simulink library "Suspension_Utilities"  (R2025a)
settings: Solver=VariableStepAuto  StartTime=0.0  StopTime=10.0  RelTol=1e-3
undefined symbols (not defined in the file or in its folder): Ac, Af, Ar, hp1, hp2, hp3, hp_in, hp_in_f_ua, hp_in_r_ua, hp_mount_subframe, hp_shk_frame, hp_spr_bot, hp_spr_top, hpb, hpf, hpo, hpx, hpz, Newton, Raphson, rotYAxis, SubframeConnection, Upper_Arm_to_Subframe, Visual, X, Y, Z
libraries: sm_lib x75, $bdroot x23, linkage_bushing_6DOF_lib x13, fl_lib x4, sharedtransformsys x3, linkage_bushing_5DOF_lib x2, nesl_utility x1
(part 3 of 3)

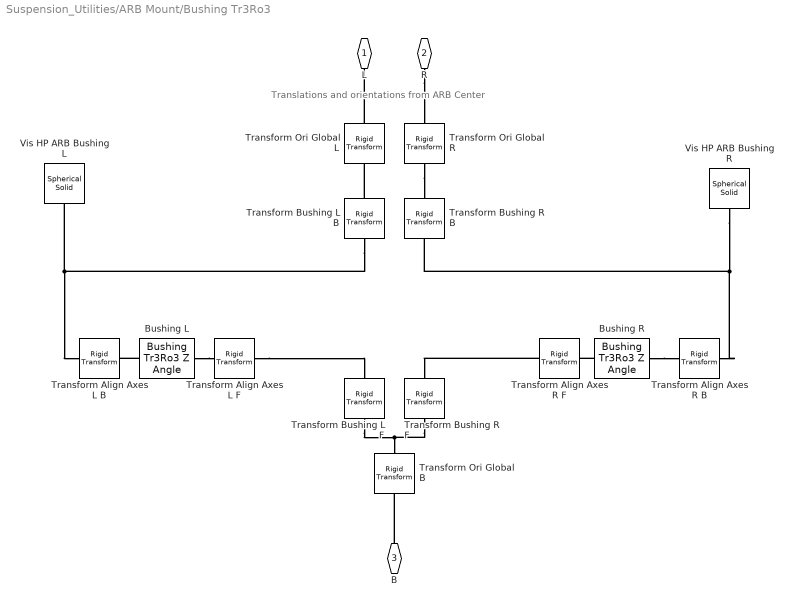
== system Suspension_Utilities/ARB Mount/Bushing Tr3Ro3 ==
  note: Translations and orientations from ARB Center
  Bushing L : linkage_bushing_6DOF_lib/Bushing Tr3Ro3 Z Angle  VariantControl=Bushing_Tr3Ro3  checkbox_setTargets=off  leftOrRight=1  qOriZ=Connection.qOriZ.Value  sprx=Connection.SpringX  spry=Connection.SpringY  sprz=Connection.SpringZ  damx=Connection.DamperX  damy=Connection.DamperY  damz=Connection.DamperZ  sprqx=Connection.SpringqX  sprqy=Connection.SpringqY  sprqz=Connection.SpringqZ  damqx=Connection.DamperqX  damqy=Connection.DamperqY  damqz=Connection.DamperqZ  shell_or=Visual.hp.rad*2  shell_len=Visual.hp.rad*2  shell_clr=Visual.BushingShell.clr  shell_opc=Visual.part.opc  sleeve_clr=Visual.Bushing.clr  sleeve_opc=Visual.part.opc
  Bushing R : linkage_bushing_6DOF_lib/Bushing Tr3Ro3 Z Angle  VariantControl=Bushing_Tr3Ro3  checkbox_setTargets=off  leftOrRight=-1  qOriZ=Connection.qOriZ.Value  sprx=Connection.SpringX  spry=Connection.SpringY  sprz=Connection.SpringZ  damx=Connection.DamperX  damy=Connection.DamperY  damz=Connection.DamperZ  sprqx=Connection.SpringqX  sprqy=Connection.SpringqY  sprqz=Connection.SpringqZ  damqx=Connection.DamperqX  damqy=Connection.DamperqY  damqz=Connection.DamperqZ  shell_or=Visual.hp.rad*2  shell_len=Visual.hp.rad*2  shell_clr=Visual.BushingShell.clr  shell_opc=Visual.part.opc  sleeve_clr=Visual.Bushing.clr  sleeve_opc=Visual.part.opc
  Transform Align Axes L B : sm_lib/Frames and Transforms/Rigid Transform  RotationMethod=RotationSequence  FollAlignAxisA=+X  BaseAlignAxisA=+Y  FollAlignAxisB=+Y  BaseAlignAxisB=+Z  RotationStandardAxis=+Z  RotationAngle=90  RotationAngleUnits=deg  RotationArbitraryAxis=[0 0 1]  RotationSequenceAxes=FollowerAxes  RotationSequence=XZX  RotationSequenceAngles=[90 0 0]  RotationSequenceAnglesUnits=deg  RotationMatrix=[1 0 0; 0 1 0; 0 0 1]  Quaternion=[1 0 0 0]  TranslationMethod=None  TranslationCartesianOffset=[0 0 0]  TranslationCartesianOffsetUnits=m  TranslationStandardAxis=+Z  TranslationStandardOffset=0  TranslationStandardOffsetUnits=m  TranslationROffset=0  TranslationROffsetUnits=m  TranslationThetaOffset=0  TranslationThetaOffsetUnits=deg  TranslationZOffset=0  TranslationZOffsetUnits=m
  Transform Align Axes L F : sm_lib/Frames and Transforms/Rigid Transform  RotationMethod=RotationSequence  FollAlignAxisA=+X  BaseAlignAxisA=+Y  FollAlignAxisB=+Y  BaseAlignAxisB=+Z  RotationStandardAxis=+Z  RotationAngle=90  RotationAngleUnits=deg  RotationArbitraryAxis=[0 0 1]  RotationSequenceAxes=FollowerAxes  RotationSequence=XZX  RotationSequenceAngles=[90 0 0]  RotationSequenceAnglesUnits=deg  RotationMatrix=[1 0 0; 0 1 0; 0 0 1]  Quaternion=[1 0 0 0]  TranslationMethod=None  TranslationCartesianOffset=[0 0 0]  TranslationCartesianOffsetUnits=m  TranslationStandardAxis=+Z  TranslationStandardOffset=0  TranslationStandardOffsetUnits=m  TranslationROffset=0  TranslationROffsetUnits=m  TranslationThetaOffset=0  TranslationThetaOffsetUnits=deg  TranslationZOffset=0  TranslationZOffsetUnits=m
  Transform Align Axes R B : sm_lib/Frames and Transforms/Rigid Transform  RotationMethod=RotationSequence  FollAlignAxisA=+X  BaseAlignAxisA=+Y  FollAlignAxisB=+Y  BaseAlignAxisB=+Z  RotationStandardAxis=+Z  RotationAngle=90  RotationAngleUnits=deg  RotationArbitraryAxis=[0 0 1]  RotationSequenceAxes=FollowerAxes  RotationSequence=XZX  RotationSequenceAngles=[90 0 0]  RotationSequenceAnglesUnits=deg  RotationMatrix=[1 0 0; 0 1 0; 0 0 1]  Quaternion=[1 0 0 0]  TranslationMethod=None  TranslationCartesianOffset=[0 0 0]  TranslationCartesianOffsetUnits=m  TranslationStandardAxis=+Z  TranslationStandardOffset=0  TranslationStandardOffsetUnits=m  TranslationROffset=0  TranslationROffsetUnits=m  TranslationThetaOffset=0  TranslationThetaOffsetUnits=deg  TranslationZOffset=0  TranslationZOffsetUnits=m
  Transform Align Axes R F : sm_lib/Frames and Transforms/Rigid Transform  RotationMethod=RotationSequence  FollAlignAxisA=+X  BaseAlignAxisA=+Y  FollAlignAxisB=+Y  BaseAlignAxisB=+Z  RotationStandardAxis=+Z  RotationAngle=90  RotationAngleUnits=deg  RotationArbitraryAxis=[0 0 1]  RotationSequenceAxes=FollowerAxes  RotationSequence=XZX  RotationSequenceAngles=[90 0 0]  RotationSequenceAnglesUnits=deg  RotationMatrix=[1 0 0; 0 1 0; 0 0 1]  Quaternion=[1 0 0 0]  TranslationMethod=None  TranslationCartesianOffset=[0 0 0]  TranslationCartesianOffsetUnits=m  TranslationStandardAxis=+Z  TranslationStandardOffset=0  TranslationStandardOffsetUnits=m  TranslationROffset=0  TranslationROffsetUnits=m  TranslationThetaOffset=0  TranslationThetaOffsetUnits=deg  TranslationZOffset=0  TranslationZOffsetUnits=m
  Transform Bushing L B : sm_lib/Frames and Transforms/Rigid Transform  RotationMethod=None  FollAlignAxisA=+X  BaseAlignAxisA=+Y  FollAlignAxisB=+Y  BaseAlignAxisB=+Z  RotationStandardAxis=+Z  RotationAngle=0.0  RotationAngleUnits=deg  RotationArbitraryAxis=[0 0 1]  RotationSequenceAxes=FollowerAxes  RotationSequence=XYX  RotationSequenceAngles=[0 0 0]  RotationSequenceAnglesUnits=deg  RotationMatrix=[1 0 0; 0 1 0; 0 0 1]  Quaternion=[1 0 0 0]  TranslationMethod=Cartesian  TranslationCartesianOffset=hp_mount_subframe-hp_in.*[1 0 1]  TranslationCartesianOffsetUnits=m  TranslationStandardAxis=+Z  TranslationStandardOffset=0  TranslationStandardOffsetUnits=m  TranslationROffset=0  TranslationROffsetUnits=m  TranslationThetaOffset=0  TranslationThetaOffsetUnits=deg  TranslationZOffset=0  TranslationZOffsetUnits=m
  Transform Bushing L F : sm_lib/Frames and Transforms/Rigid Transform  RotationMethod=None  FollAlignAxisA=+X  BaseAlignAxisA=+Y  FollAlignAxisB=+Y  BaseAlignAxisB=+Z  RotationStandardAxis=+Z  RotationAngle=0.0  RotationAngleUnits=deg  RotationArbitraryAxis=[0 0 1]  RotationSequenceAxes=FollowerAxes  RotationSequence=XYX  RotationSequenceAngles=[0 0 0]  RotationSequenceAnglesUnits=deg  RotationMatrix=[1 0 0; 0 1 0; 0 0 1]  Quaternion=[1 0 0 0]  TranslationMethod=Cartesian  TranslationCartesianOffset=hp_mount_subframe-hp_in.*[1 0 1]  TranslationCartesianOffsetUnits=m  TranslationStandardAxis=+Z  TranslationStandardOffset=0  TranslationStandardOffsetUnits=m  TranslationROffset=0  TranslationROffsetUnits=m  TranslationThetaOffset=0  TranslationThetaOffsetUnits=deg  TranslationZOffset=0  TranslationZOffsetUnits=m
  Transform Bushing R B : sm_lib/Frames and Transforms/Rigid Transform  RotationMethod=None  FollAlignAxisA=+X  BaseAlignAxisA=+Y  FollAlignAxisB=+Y  BaseAlignAxisB=+Z  RotationStandardAxis=+Z  RotationAngle=0.0  RotationAngleUnits=deg  RotationArbitraryAxis=[0 0 1]  RotationSequenceAxes=FollowerAxes  RotationSequence=XYX  RotationSequenceAngles=[0 0 0]  RotationSequenceAnglesUnits=deg  RotationMatrix=[1 0 0; 0 1 0; 0 0 1]  Quaternion=[1 0 0 0]  TranslationMethod=Cartesian  TranslationCartesianOffset=hp_mount_subframe.*[1 -1 1]-hp_in.*[1 0 1]  TranslationCartesianOffsetUnits=m  TranslationStandardAxis=+Z  TranslationStandardOffset=0  TranslationStandardOffsetUnits=m  TranslationROffset=0  TranslationROffsetUnits=m  TranslationThetaOffset=0  TranslationThetaOffsetUnits=deg  TranslationZOffset=0  TranslationZOffsetUnits=m
  Transform Bushing R F : sm_lib/Frames and Transforms/Rigid Transform  RotationMethod=None  FollAlignAxisA=+X  BaseAlignAxisA=+Y  FollAlignAxisB=+Y  BaseAlignAxisB=+Z  RotationStandardAxis=+Z  RotationAngle=0.0  RotationAngleUnits=deg  RotationArbitraryAxis=[0 0 1]  RotationSequenceAxes=FollowerAxes  RotationSequence=XYX  RotationSequenceAngles=[0 0 0]  RotationSequenceAnglesUnits=deg  RotationMatrix=[1 0 0; 0 1 0; 0 0 1]  Quaternion=[1 0 0 0]  TranslationMethod=Cartesian  TranslationCartesianOffset=hp_mount_subframe.*[1 -1 1]-hp_in.*[1 0 1]  TranslationCartesianOffsetUnits=m  TranslationStandardAxis=+Z  TranslationStandardOffset=0  TranslationStandardOffsetUnits=m  TranslationROffset=0  TranslationROffsetUnits=m  TranslationThetaOffset=0  TranslationThetaOffsetUnits=deg  TranslationZOffset=0  TranslationZOffsetUnits=m
  Transform Ori Global B : sm_lib/Frames and Transforms/Rigid Transform  RotationMethod=StandardAxis  FollAlignAxisA=+X  BaseAlignAxisA=+Y  FollAlignAxisB=+Y  BaseAlignAxisB=+Z  RotationStandardAxis=+X  RotationAngle=90  RotationAngleUnits=deg  RotationArbitraryAxis=[0 0 1]  RotationSequenceAxes=FollowerAxes  RotationSequence=XYX  RotationSequenceAngles=[0 0 0]  RotationSequenceAnglesUnits=deg  RotationMatrix=[1 0 0; 0 1 0; 0 0 1]  Quaternion=[1 0 0 0]  TranslationMethod=None  TranslationCartesianOffset=[0 0 0]  TranslationCartesianOffsetUnits=m  TranslationStandardAxis=+Z  TranslationStandardOffset=0  TranslationStandardOffsetUnits=m  TranslationROffset=0  TranslationROffsetUnits=m  TranslationThetaOffset=0  TranslationThetaOffsetUnits=deg  TranslationZOffset=0  TranslationZOffsetUnits=m
  Transform Ori Global L : sm_lib/Frames and Transforms/Rigid Transform  RotationMethod=StandardAxis  FollAlignAxisA=+X  BaseAlignAxisA=+Y  FollAlignAxisB=+Y  BaseAlignAxisB=+Z  RotationStandardAxis=+X  RotationAngle=90  RotationAngleUnits=deg  RotationArbitraryAxis=[0 0 1]  RotationSequenceAxes=FollowerAxes  RotationSequence=XYX  RotationSequenceAngles=[0 0 0]  RotationSequenceAnglesUnits=deg  RotationMatrix=[1 0 0; 0 1 0; 0 0 1]  Quaternion=[1 0 0 0]  TranslationMethod=None  TranslationCartesianOffset=[0 0 0]  TranslationCartesianOffsetUnits=m  TranslationStandardAxis=+Z  TranslationStandardOffset=0  TranslationStandardOffsetUnits=m  TranslationROffset=0  TranslationROffsetUnits=m  TranslationThetaOffset=0  TranslationThetaOffsetUnits=deg  TranslationZOffset=0  TranslationZOffsetUnits=m
  Transform Ori Global R : sm_lib/Frames and Transforms/Rigid Transform  RotationMethod=StandardAxis  FollAlignAxisA=+X  BaseAlignAxisA=+Y  FollAlignAxisB=+Y  BaseAlignAxisB=+Z  RotationStandardAxis=+X  RotationAngle=90  RotationAngleUnits=deg  RotationArbitraryAxis=[0 0 1]  RotationSequenceAxes=FollowerAxes  RotationSequence=XYX  RotationSequenceAngles=[0 0 0]  RotationSequenceAnglesUnits=deg  RotationMatrix=[1 0 0; 0 1 0; 0 0 1]  Quaternion=[1 0 0 0]  TranslationMethod=None  TranslationCartesianOffset=[0 0 0]  TranslationCartesianOffsetUnits=m  TranslationStandardAxis=+Z  TranslationStandardOffset=0  TranslationStandardOffsetUnits=m  TranslationROffset=0  TranslationROffsetUnits=m  TranslationThetaOffset=0  TranslationThetaOffsetUnits=deg  TranslationZOffset=0  TranslationZOffsetUnits=m
  Vis HP ARB Bushing L : sm_lib/Body Elements/Spherical Solid  SphereRadius=rad_hp  SphereRadiusUnits=m  ExportEntireGeometry=off  InertiaType=CalculateFromGeometry  BasedOnType=Density  Density=1000  DensityUnits=kg/m^3  Mass=1  MassUnits=kg  CenterOfMass=[0 0 0]  CenterOfMassUnits=m  MomentsOfInertia=[1 1 1]  MomentsOfInertiaUnits=kg*m^2  ProductsOfInertia=[0 0 0]  ProductsOfInertiaUnits=kg*m^2  GraphicType=FromGeometry  MarkerShape=Sphere  MarkerSize=10  GraphicVisPropType=SimpleVisualProperties  GraphicDiffuseColor=clr_hp  GraphicOpacity=opc_hp  GraphicSpecularColor=[0.5 0.5 0.5 1.0]  GraphicAmbientColor=[0.15 0.15 0.15 1.0]  GraphicEmissiveColor=[0.0 0.0 0.0 1.0]  GraphicShininess=75  DoExposeReferenceFrame=on  SerializedFrames=<Frames/>
  Vis HP ARB Bushing R : sm_lib/Body Elements/Spherical Solid  SphereRadius=rad_hp  SphereRadiusUnits=m  ExportEntireGeometry=off  InertiaType=CalculateFromGeometry  BasedOnType=Density  Density=1000  DensityUnits=kg/m^3  Mass=1  MassUnits=kg  CenterOfMass=[0 0 0]  CenterOfMassUnits=m  MomentsOfInertia=[1 1 1]  MomentsOfInertiaUnits=kg*m^2  ProductsOfInertia=[0 0 0]  ProductsOfInertiaUnits=kg*m^2  GraphicType=FromGeometry  MarkerShape=Sphere  MarkerSize=10  GraphicVisPropType=SimpleVisualProperties  GraphicDiffuseColor=clr_hp  GraphicOpacity=opc_hp  GraphicSpecularColor=[0.5 0.5 0.5 1.0]  GraphicAmbientColor=[0.15 0.15 0.15 1.0]  GraphicEmissiveColor=[0.0 0.0 0.0 1.0]  GraphicShininess=75  DoExposeReferenceFrame=on  SerializedFrames=<Frames/>
  L : PMIOPort  Side=Right
  R : PMIOPort  Port=2  Side=Right
  B : PMIOPort  Port=3  Side=Left
  connections:
  Transform Bushing L B/LConn1 -- Transform Ori Global L/RConn1
  Transform Ori Global L/LConn1 -- L/RConn1
  Transform Align Axes L F/LConn1 -- Transform Bushing L F/RConn1
  Transform Ori Global B/RConn1 -- Transform Bushing R F/LConn1 -- Transform Bushing L F/LConn1
  Transform Align Axes R F/LConn1 -- Transform Bushing R F/RConn1
  B/RConn1 -- Transform Ori Global B/LConn1
  Transform Ori Global R/RConn1 -- Transform Bushing R B/LConn1
  Vis HP ARB Bushing L/RConn1 -- Transform Align Axes L B/LConn1 -- Transform Bushing L B/RConn1
  Transform Bushing R B/RConn1 -- Transform Align Axes R B/LConn1 -- Vis HP ARB Bushing R/RConn1
  R/RConn1 -- Transform Ori Global R/LConn1
  Bushing R/LConn1 -- Transform Align Axes R B/RConn1
  Bushing R/RConn1 -- Transform Align Axes R F/RConn1
  Bushing L/LConn1 -- Transform Align Axes L B/RConn1
  Bushing L/RConn1 -- Transform Align Axes L F/RConn1

== system Suspension_Utilities/ARB Mount/Rigid 1Rev ==
  Revolute ARB Mount : sm_lib/Joints/Revolute Joint  JointMode=Normal  CompositeWrenchDir=FollowerOnBase  CompositeWrenchFrame=BaseFrame  SenseConstraintForce=off  SenseConstraintTorque=off  SenseTotalForce=off  SenseTotalTorque=off  PositionTargetSpecify=on  PositionTargetPriority=Low  PositionTargetValue=0  PositionTargetValueUnits=deg  VelocityTargetSpecify=off  VelocityTargetPriority=High  VelocityTargetValue=0  VelocityTargetValueUnits=deg/s  EquilibriumPosition=0  EquilibriumPositionUnits=deg  SpringStiffness=0  SpringStiffnessUnits=N*m/deg  DampingCoefficient=0  DampingCoefficientUnits=N*m/(deg/s)  LowerLimitSpecify=off  LowerLimitBound=-90  LowerLimitBoundUnits=deg  LowerLimitStiffness=1e4  LowerLimitStiffnessUnits=N*m/deg  LowerLimitDamping=10  LowerLimitDampingUnits=N*m/(deg/s)  LowerLimitTransitionRegionWidth=0.1  LowerLimitTransitionRegionWidthUnits=deg  UpperLimitSpecify=off  UpperLimitBound=90  UpperLimitBoundUnits=deg  UpperLimitStiffness=1e4  UpperLimitStiffnessUnits=N*m/deg  UpperLimitDamping=10  UpperLimitDampingUnits=N*m/(deg/s)  UpperLimitTransitionRegionWidth=0.1  UpperLimitTransitionRegionWidthUnits=deg  TorqueActuationMode=NoTorque  MotionActuationMode=ComputedMotion  SensePosition=off  SenseVelocity=off  SenseAcceleration=off  SenseTorqueForce=off  SenseLowerLimitTorqueForce=off  SenseUpperLimitTorqueForce=off
  L : PMIOPort  Side=Right
  R : PMIOPort  Port=2  Side=Right
  B : PMIOPort  Port=3  Side=Left
  connections:
  Revolute ARB Mount/LConn1 -- B/RConn1
  Revolute ARB Mount/RConn1 -- R/RConn1

== system Suspension_Utilities/Arm to Subframe Revolute/Bushing Ax3 ==
  Bushing Af : linkage_bushing_6DOF_lib/Bushing Ax3  VariantControl=Bushing_Ax3  checkbox_setTargets=on  leftOrRight=rhs_y  hp_j=hp_f  hp_z=Connection.sFAxialOrientationZ.Value  hp_x=Connection.sFAxialOrientationX.Value  AxisAttachment=Connection.AxisAttachment.class.Value  sprx=Connection.FSpringX  spry=Connection.FSpringY  sprz=Connection.FSpringZ  damx=Connection.FDamperX  damy=Connection.FDamperY  damz=Connection.FDamperZ  shell_or=Visual.hp.rad*2  shell_len=Visual.hp.rad*2  shell_clr=Visual.BushingShell.clr  shell_opc=Visual.part.opc  sleeve_clr=Visual.Bushing.clr  sleeve_opc=Visual.part.opc
  Bushing Ar : linkage_bushing_6DOF_lib/Bushing Ax3  VariantControl=Bushing_Ax3  checkbox_setTargets=off  leftOrRight=rhs_y  hp_j=hp_r  hp_z=Connection.sRAxialOrientationZ.Value  hp_x=Connection.sRAxialOrientationX.Value  AxisAttachment=Connection.AxisAttachment.class.Value  sprx=Connection.RSpringX  spry=Connection.RSpringY  sprz=Connection.RSpringZ  damx=Connection.RDamperX  damy=Connection.RDamperY  damz=Connection.RDamperZ  shell_or=Visual.hp.rad*2  shell_len=Visual.hp.rad*2  shell_clr=Visual.BushingShell.clr  shell_opc=Visual.part.opc  sleeve_clr=Visual.Bushing.clr  sleeve_opc=Visual.part.opc
  Simscape Bus : SimscapeBus  HierarchyStrings=Af;Ac;Ar
  Simscape Bus1 : SimscapeBus  HierarchyStrings=Af;Ac;Ar
  Terminator UAc Body : $bdroot/Terminator  SystemSampleTime=-1  VariantActivationTime=update diagram  EmptyChoice=off  PassThrough=off  PassThroughVariantControl=(default)  EmptyChoiceVariantControl=(default)  AllowFlexibleInterface=on  Latency=0  AutoFrameSizeCalculation=off
  Terminator UAc Chassis : $bdroot/Terminator  SystemSampleTime=-1  VariantActivationTime=update diagram  EmptyChoice=off  PassThrough=off  PassThroughVariantControl=(default)  EmptyChoiceVariantControl=(default)  AllowFlexibleInterface=on  Latency=0  AutoFrameSizeCalculation=off
  F : PMIOPort  Side=Right
  " B" : PMIOPort  Port=2  Side=Left
  connections:
  Simscape Bus1/RConn1 -- F/RConn1
  Simscape Bus/RConn1 -- " B"/RConn1
  Bushing Af/LConn1 -- Simscape Bus/LConn1
  Bushing Ar/LConn1 -- Simscape Bus/LConn3
  Simscape Bus1/LConn1 -- Bushing Af/RConn1
  Simscape Bus1/LConn3 -- Bushing Ar/RConn1
  Terminator UAc Body/RConn1 -- Simscape Bus/LConn2
  Terminator UAc Chassis/RConn1 -- Simscape Bus1/LConn2

== system Suspension_Utilities/Arm to Subframe Revolute/Bushing AxRad ==
  Bushing Af : linkage_bushing_6DOF_lib/Bushing AxRad  VariantControl=Bushing_AxRad  checkbox_setTargets=on  leftOrRight=rhs_y  hp_j=hp_f  hp_z=hp_r  sprRad=Connection.RadialSpring  damRad=Connection.RadialDamper  sprAxi=Connection.AxialSpring  damAxi=Connection.AxialDamper  shell_or=Visual.hp.rad*2  shell_len=Visual.hp.rad*2  shell_clr=Visual.BushingShell.clr  shell_opc=Visual.part.opc  sleeve_clr=Visual.Bushing.clr  sleeve_opc=Visual.part.opc
  Bushing Ar : linkage_bushing_6DOF_lib/Bushing AxRad  VariantControl=Bushing_AxRad  checkbox_setTargets=off  leftOrRight=rhs_y  hp_j=hp_r  hp_z=hp_f  sprRad=Connection.RadialSpring  damRad=Connection.RadialDamper  sprAxi=Connection.AxialSpring  damAxi=Connection.AxialDamper  shell_or=Visual.hp.rad*2  shell_len=Visual.hp.rad*2  shell_clr=Visual.BushingShell.clr  shell_opc=Visual.part.opc  sleeve_clr=Visual.Bushing.clr  sleeve_opc=Visual.part.opc
  Simscape Bus : SimscapeBus  HierarchyStrings=Af;Ac;Ar
  Simscape Bus1 : SimscapeBus  HierarchyStrings=Af;Ac;Ar
  Terminator UAc Body : $bdroot/Terminator  SystemSampleTime=-1  VariantActivationTime=update diagram  EmptyChoice=off  PassThrough=off  PassThroughVariantControl=(default)  EmptyChoiceVariantControl=(default)  AllowFlexibleInterface=on  Latency=0  AutoFrameSizeCalculation=off
  Terminator UAc Chassis : $bdroot/Terminator  SystemSampleTime=-1  VariantActivationTime=update diagram  EmptyChoice=off  PassThrough=off  PassThroughVariantControl=(default)  EmptyChoiceVariantControl=(default)  AllowFlexibleInterface=on  Latency=0  AutoFrameSizeCalculation=off
  F : PMIOPort  Side=Right
  " B" : PMIOPort  Port=2  Side=Left
  connections:
  Terminator UAc Chassis/RConn1 -- Simscape Bus1/LConn2
  Terminator UAc Body/RConn1 -- Simscape Bus/LConn2
  Simscape Bus/RConn1 -- " B"/RConn1
  Simscape Bus1/RConn1 -- F/RConn1
  Bushing Af/LConn1 -- Simscape Bus/LConn1
  Bushing Af/RConn1 -- Simscape Bus1/LConn1
  Bushing Ar/LConn1 -- Simscape Bus/LConn3
  Bushing Ar/RConn1 -- Simscape Bus1/LConn3

== system Suspension_Utilities/Arm to Subframe Revolute/Bushing Tr3Ro3 ==
  Bushing Af : linkage_bushing_6DOF_lib/Bushing Tr3Ro3 2Pts  VariantControl=Bushing_Tr3Ro3  checkbox_setTargets=on  leftOrRight=rhs_y  hp_j=hp_f  hp_z=Connection.sFAxialOrientationZ.Value  hp_x=Connection.sFAxialOrientationX.Value  sprx=Connection.FSpringX  spry=Connection.FSpringY  sprz=Connection.FSpringZ  damx=Connection.FDamperX  damy=Connection.FDamperY  damz=Connection.FDamperZ  sprqx=Connection.FSpringqX  sprqy=Connection.FSpringqY  sprqz=Connection.FSpringqZ  damqx=Connection.FDamperqX  damqy=Connection.FDamperqY  damqz=Connection.FDamperqZ  shell_or=Visual.hp.rad*2  shell_len=Visual.hp.rad*2  shell_clr=Visual.BushingShell.clr  shell_opc=Visual.part.opc  sleeve_clr=Visual.Bushing.clr  sleeve_opc=Visual.part.opc
  Bushing Ar : linkage_bushing_6DOF_lib/Bushing Tr3Ro3 2Pts  VariantControl=Bushing_Tr3Ro3  checkbox_setTargets=off  leftOrRight=rhs_y  hp_j=hp_r  hp_z=Connection.sRAxialOrientationZ.Value  hp_x=Connection.sRAxialOrientationX.Value  sprx=Connection.RSpringX  spry=Connection.RSpringY  sprz=Connection.RSpringZ  damx=Connection.RDamperX  damy=Connection.RDamperY  damz=Connection.RDamperZ  sprqx=Connection.RSpringqX  sprqy=Connection.RSpringqY  sprqz=Connection.RSpringqZ  damqx=Connection.RDamperqX  damqy=Connection.RDamperqY  damqz=Connection.RDamperqZ  shell_or=Visual.hp.rad*2  shell_len=Visual.hp.rad*2  shell_clr=Visual.BushingShell.clr  shell_opc=Visual.part.opc  sleeve_clr=Visual.Bushing.clr  sleeve_opc=Visual.part.opc
  Simscape Bus : SimscapeBus  HierarchyStrings=Af;Ac;Ar
  Simscape Bus1 : SimscapeBus  HierarchyStrings=Af;Ac;Ar
  Terminator UAc Body : $bdroot/Terminator  SystemSampleTime=-1  VariantActivationTime=update diagram  EmptyChoice=off  PassThrough=off  PassThroughVariantControl=(default)  EmptyChoiceVariantControl=(default)  AllowFlexibleInterface=on  Latency=0  AutoFrameSizeCalculation=off
  Terminator UAc Chassis : $bdroot/Terminator  SystemSampleTime=-1  VariantActivationTime=update diagram  EmptyChoice=off  PassThrough=off  PassThroughVariantControl=(default)  EmptyChoiceVariantControl=(default)  AllowFlexibleInterface=on  Latency=0  AutoFrameSizeCalculation=off
  F : PMIOPort  Side=Right
  " B" : PMIOPort  Port=2  Side=Left
  connections:
  Terminator UAc Chassis/RConn1 -- Simscape Bus1/LConn2
  Terminator UAc Body/RConn1 -- Simscape Bus/LConn2
  Simscape Bus/RConn1 -- " B"/RConn1
  Simscape Bus1/RConn1 -- F/RConn1
  Bushing Af/LConn1 -- Simscape Bus/LConn1
  Bushing Af/RConn1 -- Simscape Bus1/LConn1
  Bushing Ar/RConn1 -- Simscape Bus1/LConn3
  Bushing Ar/LConn1 -- Simscape Bus/LConn3

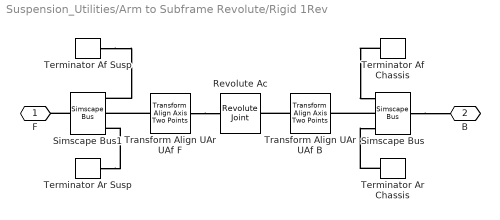
== system Suspension_Utilities/Arm to Subframe Revolute/Rigid 1Rev ==
  Revolute Ac : sm_lib/Joints/Revolute Joint  JointMode=Normal  CompositeWrenchDir=FollowerOnBase  CompositeWrenchFrame=BaseFrame  SenseConstraintForce=off  SenseConstraintTorque=off  SenseTotalForce=off  SenseTotalTorque=off  PositionTargetSpecify=on  PositionTargetPriority=Low  PositionTargetValue=0  PositionTargetValueUnits=deg  VelocityTargetSpecify=off  VelocityTargetPriority=High  VelocityTargetValue=0  VelocityTargetValueUnits=deg/s  EquilibriumPosition=0  EquilibriumPositionUnits=deg  SpringStiffness=0  SpringStiffnessUnits=N*m/deg  DampingCoefficient=0  DampingCoefficientUnits=N*m/(deg/s)  LowerLimitSpecify=off  LowerLimitBound=-90  LowerLimitBoundUnits=deg  LowerLimitStiffness=1e4  LowerLimitStiffnessUnits=N*m/deg  LowerLimitDamping=10  LowerLimitDampingUnits=N*m/(deg/s)  LowerLimitTransitionRegionWidth=0.1  LowerLimitTransitionRegionWidthUnits=deg  UpperLimitSpecify=off  UpperLimitBound=90  UpperLimitBoundUnits=deg  UpperLimitStiffness=1e4  UpperLimitStiffnessUnits=N*m/deg  UpperLimitDamping=10  UpperLimitDampingUnits=N*m/(deg/s)  UpperLimitTransitionRegionWidth=0.1  UpperLimitTransitionRegionWidthUnits=deg  TorqueActuationMode=NoTorque  MotionActuationMode=ComputedMotion  SensePosition=off  SenseVelocity=off  SenseAcceleration=off  SenseTorqueForce=off  SenseLowerLimitTorqueForce=off  SenseUpperLimitTorqueForce=off
  Simscape Bus : SimscapeBus  HierarchyStrings=Af;Ac;Ar
  Simscape Bus1 : SimscapeBus  HierarchyStrings=Af;Ac;Ar
  Terminator Af Chassis : $bdroot/Terminator  SystemSampleTime=-1  VariantActivationTime=update diagram  EmptyChoice=off  PassThrough=off  PassThroughVariantControl=(default)  EmptyChoiceVariantControl=(default)  AllowFlexibleInterface=on  Latency=0  AutoFrameSizeCalculation=off
  Terminator Af Susp : $bdroot/Terminator  SystemSampleTime=-1  VariantActivationTime=update diagram  EmptyChoice=off  PassThrough=off  PassThroughVariantControl=(default)  EmptyChoiceVariantControl=(default)  AllowFlexibleInterface=on  Latency=0  AutoFrameSizeCalculation=off
  Terminator Ar Chassis : $bdroot/Terminator  SystemSampleTime=-1  VariantActivationTime=update diagram  EmptyChoice=off  PassThrough=off  PassThroughVariantControl=(default)  EmptyChoiceVariantControl=(default)  AllowFlexibleInterface=on  Latency=0  AutoFrameSizeCalculation=off
  Terminator Ar Susp : $bdroot/Terminator  SystemSampleTime=-1  VariantActivationTime=update diagram  EmptyChoice=off  PassThrough=off  PassThroughVariantControl=(default)  EmptyChoiceVariantControl=(default)  AllowFlexibleInterface=on  Latency=0  AutoFrameSizeCalculation=off
  Transform Align UAr UAf B : $bdroot/Transform Align Axis Two Points  hp_b=hp_r.*rhs_hp  hp_t=hp_f.*rhs_hp  popup_f_axis=+Z
  Transform Align UAr UAf F : $bdroot/Transform Align Axis Two Points  hp_b=hp_r.*rhs_hp  hp_t=hp_f.*rhs_hp  popup_f_axis=+Z
  F : PMIOPort  Side=Right
  " B" : PMIOPort  Port=2  Side=Left
  connections:
  Transform Align UAr UAf F/LConn1 -- Simscape Bus1/LConn2
  Transform Align UAr UAf B/RConn1 -- Revolute Ac/LConn1
  Simscape Bus/LConn2 -- Transform Align UAr UAf B/LConn1
  Transform Align UAr UAf F/RConn1 -- Revolute Ac/RConn1
  Simscape Bus/RConn1 -- " B"/RConn1
  Simscape Bus1/RConn1 -- F/RConn1
  Terminator Af Susp/RConn1 -- Simscape Bus1/LConn1
  Terminator Ar Susp/RConn1 -- Simscape Bus1/LConn3
  Terminator Af Chassis/RConn1 -- Simscape Bus/LConn1
  Terminator Ar Chassis/RConn1 -- Simscape Bus/LConn3

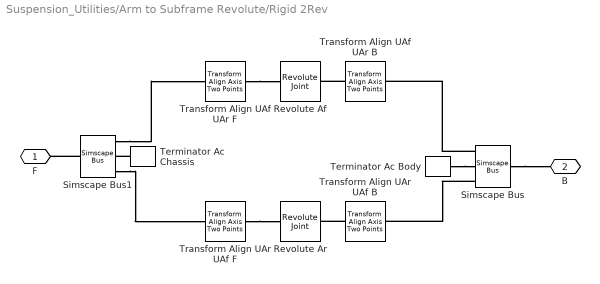
== system Suspension_Utilities/Arm to Subframe Revolute/Rigid 2Rev ==
  Revolute Af : sm_lib/Joints/Revolute Joint  JointMode=Normal  CompositeWrenchDir=FollowerOnBase  CompositeWrenchFrame=BaseFrame  SenseConstraintForce=off  SenseConstraintTorque=off  SenseTotalForce=off  SenseTotalTorque=off  PositionTargetSpecify=on  PositionTargetPriority=Low  PositionTargetValue=0  PositionTargetValueUnits=deg  VelocityTargetSpecify=off  VelocityTargetPriority=High  VelocityTargetValue=0  VelocityTargetValueUnits=deg/s  EquilibriumPosition=0  EquilibriumPositionUnits=deg  SpringStiffness=0  SpringStiffnessUnits=N*m/deg  DampingCoefficient=0  DampingCoefficientUnits=N*m/(deg/s)  LowerLimitSpecify=off  LowerLimitBound=-90  LowerLimitBoundUnits=deg  LowerLimitStiffness=1e4  LowerLimitStiffnessUnits=N*m/deg  LowerLimitDamping=10  LowerLimitDampingUnits=N*m/(deg/s)  LowerLimitTransitionRegionWidth=0.1  LowerLimitTransitionRegionWidthUnits=deg  UpperLimitSpecify=off  UpperLimitBound=90  UpperLimitBoundUnits=deg  UpperLimitStiffness=1e4  UpperLimitStiffnessUnits=N*m/deg  UpperLimitDamping=10  UpperLimitDampingUnits=N*m/(deg/s)  UpperLimitTransitionRegionWidth=0.1  UpperLimitTransitionRegionWidthUnits=deg  TorqueActuationMode=NoTorque  MotionActuationMode=ComputedMotion  SensePosition=off  SenseVelocity=off  SenseAcceleration=off  SenseTorqueForce=off  SenseLowerLimitTorqueForce=off  SenseUpperLimitTorqueForce=off
  Revolute Ar : sm_lib/Joints/Revolute Joint  JointMode=Normal  CompositeWrenchDir=FollowerOnBase  CompositeWrenchFrame=BaseFrame  SenseConstraintForce=off  SenseConstraintTorque=off  SenseTotalForce=off  SenseTotalTorque=off  PositionTargetSpecify=off  PositionTargetPriority=Low  PositionTargetValue=0  PositionTargetValueUnits=deg  VelocityTargetSpecify=off  VelocityTargetPriority=High  VelocityTargetValue=0  VelocityTargetValueUnits=deg/s  EquilibriumPosition=0  EquilibriumPositionUnits=deg  SpringStiffness=0  SpringStiffnessUnits=N*m/deg  DampingCoefficient=0  DampingCoefficientUnits=N*m/(deg/s)  LowerLimitSpecify=off  LowerLimitBound=-90  LowerLimitBoundUnits=deg  LowerLimitStiffness=1e4  LowerLimitStiffnessUnits=N*m/deg  LowerLimitDamping=10  LowerLimitDampingUnits=N*m/(deg/s)  LowerLimitTransitionRegionWidth=0.1  LowerLimitTransitionRegionWidthUnits=deg  UpperLimitSpecify=off  UpperLimitBound=90  UpperLimitBoundUnits=deg  UpperLimitStiffness=1e4  UpperLimitStiffnessUnits=N*m/deg  UpperLimitDamping=10  UpperLimitDampingUnits=N*m/(deg/s)  UpperLimitTransitionRegionWidth=0.1  UpperLimitTransitionRegionWidthUnits=deg  TorqueActuationMode=NoTorque  MotionActuationMode=ComputedMotion  SensePosition=off  SenseVelocity=off  SenseAcceleration=off  SenseTorqueForce=off  SenseLowerLimitTorqueForce=off  SenseUpperLimitTorqueForce=off
  Simscape Bus : SimscapeBus  HierarchyStrings=Af;Ac;Ar
  Simscape Bus1 : SimscapeBus  HierarchyStrings=Af;Ac;Ar
  Terminator Ac Body : $bdroot/Terminator  SystemSampleTime=-1  VariantActivationTime=update diagram  EmptyChoice=off  PassThrough=off  PassThroughVariantControl=(default)  EmptyChoiceVariantControl=(default)  AllowFlexibleInterface=on  Latency=0  AutoFrameSizeCalculation=off
  Terminator Ac Chassis : $bdroot/Terminator  SystemSampleTime=-1  VariantActivationTime=update diagram  EmptyChoice=off  PassThrough=off  PassThroughVariantControl=(default)  EmptyChoiceVariantControl=(default)  AllowFlexibleInterface=on  Latency=0  AutoFrameSizeCalculation=off
  Transform Align UAf UAr B : $bdroot/Transform Align Axis Two Points  hp_b=hp_f.*rhs_hp  hp_t=hp_r.*rhs_hp  popup_f_axis=-Z
  Transform Align UAf UAr F : $bdroot/Transform Align Axis Two Points  hp_b=hp_f.*rhs_hp  hp_t=hp_r.*rhs_hp  popup_f_axis=-Z
  Transform Align UAr UAf B : $bdroot/Transform Align Axis Two Points  hp_b=hp_r.*rhs_hp  hp_t=hp_f.*rhs_hp  popup_f_axis=+Z
  Transform Align UAr UAf F : $bdroot/Transform Align Axis Two Points  hp_b=hp_r.*rhs_hp  hp_t=hp_f.*rhs_hp  popup_f_axis=+Z
  F : PMIOPort  Side=Right
  " B" : PMIOPort  Port=2  Side=Left
  connections:
  Simscape Bus1/LConn1 -- Transform Align UAf UAr F/LConn1
  Transform Align UAr UAf F/RConn1 -- Revolute Ar/RConn1
  Transform Align UAr UAf B/RConn1 -- Revolute Ar/LConn1
  Transform Align UAf UAr F/RConn1 -- Revolute Af/RConn1
  Transform Align UAf UAr B/RConn1 -- Revolute Af/LConn1
  Terminator Ac Body/RConn1 -- Simscape Bus/LConn2
  Terminator Ac Chassis/RConn1 -- Simscape Bus1/LConn2
  Simscape Bus1/RConn1 -- F/RConn1
  Simscape Bus/RConn1 -- " B"/RConn1
  Simscape Bus/LConn1 -- Transform Align UAf UAr B/LConn1
  Simscape Bus/LConn3 -- Transform Align UAr UAf B/LConn1
  Simscape Bus1/LConn3 -- Transform Align UAr UAf F/LConn1

== system Suspension_Utilities/Arm to Subframe Universal/Rigid UJ ==
  Transform Align Y Up In : sm_lib/Frames and Transforms/Rigid Transform  RotationMethod=StandardAxis  FollAlignAxisA=+X  BaseAlignAxisA=+Y  FollAlignAxisB=+Y  BaseAlignAxisB=+Z  RotationStandardAxis=+X  RotationAngle=90  RotationAngleUnits=deg  RotationArbitraryAxis=[0 0 1]  RotationSequenceAxes=FollowerAxes  RotationSequence=XYX  RotationSequenceAngles=[0 0 0]  RotationSequenceAnglesUnits=deg  RotationMatrix=[1 0 0; 0 1 0; 0 0 1]  Quaternion=[1 0 0 0]  TranslationMethod=None  TranslationCartesianOffset=[0 0 0]  TranslationCartesianOffsetUnits=m  TranslationStandardAxis=+Z  TranslationStandardOffset=0  TranslationStandardOffsetUnits=m  TranslationROffset=0  TranslationROffsetUnits=m  TranslationThetaOffset=0  TranslationThetaOffsetUnits=deg  TranslationZOffset=0  TranslationZOffsetUnits=m
  Transform Align Y Up Out : sm_lib/Frames and Transforms/Rigid Transform  RotationMethod=StandardAxis  FollAlignAxisA=+X  BaseAlignAxisA=+Y  FollAlignAxisB=+Y  BaseAlignAxisB=+Z  RotationStandardAxis=+X  RotationAngle=90  RotationAngleUnits=deg  RotationArbitraryAxis=[0 0 1]  RotationSequenceAxes=FollowerAxes  RotationSequence=XYX  RotationSequenceAngles=[0 0 0]  RotationSequenceAnglesUnits=deg  RotationMatrix=[1 0 0; 0 1 0; 0 0 1]  Quaternion=[1 0 0 0]  TranslationMethod=None  TranslationCartesianOffset=[0 0 0]  TranslationCartesianOffsetUnits=m  TranslationStandardAxis=+Z  TranslationStandardOffset=0  TranslationStandardOffsetUnits=m  TranslationROffset=0  TranslationROffsetUnits=m  TranslationThetaOffset=0  TranslationThetaOffsetUnits=deg  TranslationZOffset=0  TranslationZOffsetUnits=m
  Universal Joint : sm_lib/Joints/Universal Joint  JointMode=Normal  CompositeWrenchDir=FollowerOnBase  CompositeWrenchFrame=BaseFrame  SenseConstraintForce=off  SenseConstraintTorque=off  SenseTotalForce=off  SenseTotalTorque=off  RxPositionTargetSpecify=on  RxPositionTargetPriority=Low  RxPositionTargetValue=0  RxPositionTargetValueUnits=deg  RxVelocityTargetSpecify=off  RxVelocityTargetPriority=High  RxVelocityTargetValue=0  RxVelocityTargetValueUnits=deg/s  RxEquilibriumPosition=0  RxEquilibriumPositionUnits=deg  RxSpringStiffness=0  RxSpringStiffnessUnits=N*m/deg  RxDampingCoefficient=0  RxDampingCoefficientUnits=N*m/(deg/s)  RxLowerLimitSpecify=off  RxLowerLimitBound=-90  RxLowerLimitBoundUnits=deg  RxLowerLimitStiffness=1e4  RxLowerLimitStiffnessUnits=N*m/deg  RxLowerLimitDamping=10  RxLowerLimitDampingUnits=N*m/(deg/s)  RxLowerLimitTransitionRegionWidth=0.1  RxLowerLimitTransitionRegionWidthUnits=deg  RxUpperLimitSpecify=off  RxUpperLimitBound=90  RxUpperLimitBoundUnits=deg  RxUpperLimitStiffness=1e4  RxUpperLimitStiffnessUnits=N*m/deg  RxUpperLimitDamping=10  RxUpperLimitDampingUnits=N*m/(deg/s)  RxUpperLimitTransitionRegionWidth=0.1  RxUpperLimitTransitionRegionWidthUnits=deg  RxTorqueActuationMode=NoTorque  RxMotionActuationMode=ComputedMotion  RxSensePosition=off  RxSenseVelocity=off  RxSenseAcceleration=off  RxSenseTorqueForce=off  RxSenseLowerLimitTorqueForce=off  RxSenseUpperLimitTorqueForce=off  RyPositionTargetSpecify=on  RyPositionTargetPriority=High  RyPositionTargetValue=0  RyPositionTargetValueUnits=deg  RyVelocityTargetSpecify=off  RyVelocityTargetPriority=High  RyVelocityTargetValue=0  RyVelocityTargetValueUnits=deg/s  RyEquilibriumPosition=0  RyEquilibriumPositionUnits=deg  RySpringStiffness=0  RySpringStiffnessUnits=N*m/deg  RyDampingCoefficient=0  RyDampingCoefficientUnits=N*m/(deg/s)  RyLowerLimitSpecify=off  RyLowerLimitBound=-90  RyLowerLimitBoundUnits=deg  RyLowerLimitStiffness=1e4  RyLowerLimitStiffnessUnits=N*m/deg  RyLowerLimitDamping=10  RyLowerLimitDampingUnits=N*m/(deg/s)  RyLowerLimitTransitionRegionWidth=0.1  RyLowerLimitTransitionRegionWidthUnits=deg  RyUpperLimitSpecify=off  RyUpperLimitBound=90  RyUpperLimitBoundUnits=deg  RyUpperLimitStiffness=1e4  RyUpperLimitStiffnessUnits=N*m/deg  RyUpperLimitDamping=10  RyUpperLimitDampingUnits=N*m/(deg/s)  RyUpperLimitTransitionRegionWidth=0.1  RyUpperLimitTransitionRegionWidthUnits=deg  RyTorqueActuationMode=NoTorque  RyMotionActuationMode=ComputedMotion  RySensePosition=off  RySenseVelocity=off  RySenseAcceleration=off  RySenseTorqueForce=off  RySenseLowerLimitTorqueForce=off  RySenseUpperLimitTorqueForce=off
  F : PMIOPort  Side=Right
  B : PMIOPort  Port=2  Side=Left
  connections:
  B/RConn1 -- Transform Align Y Up In/LConn1
  F/RConn1 -- Transform Align Y Up Out/LConn1
  Transform Align Y Up Out/RConn1 -- Universal Joint/RConn1
  Transform Align Y Up In/RConn1 -- Universal Joint/LConn1

== system Suspension_Utilities/Bushing Align 2Pts Gimbal/Rigid Gimbal ==
  Gimbal HP Spring : sm_lib/Joints/Gimbal Joint  JointMode=Normal  CompositeWrenchDir=FollowerOnBase  CompositeWrenchFrame=BaseFrame  SenseConstraintForce=off  SenseConstraintTorque=off  SenseTotalForce=off  SenseTotalTorque=off  RxPositionTargetSpecify=off  RxPositionTargetPriority=Low  RxPositionTargetValue=0  RxPositionTargetValueUnits=deg  RxVelocityTargetSpecify=off  RxVelocityTargetPriority=High  RxVelocityTargetValue=0  RxVelocityTargetValueUnits=deg/s  RxEquilibriumPosition=0  RxEquilibriumPositionUnits=deg  RxSpringStiffness=0  RxSpringStiffnessUnits=N*m/deg  RxDampingCoefficient=0  RxDampingCoefficientUnits=N*m/(deg/s)  RxLowerLimitSpecify=off  RxLowerLimitBound=-90  RxLowerLimitBoundUnits=deg  RxLowerLimitStiffness=1e4  RxLowerLimitStiffnessUnits=N*m/deg  RxLowerLimitDamping=10  RxLowerLimitDampingUnits=N*m/(deg/s)  RxLowerLimitTransitionRegionWidth=0.1  RxLowerLimitTransitionRegionWidthUnits=deg  RxUpperLimitSpecify=off  RxUpperLimitBound=90  RxUpperLimitBoundUnits=deg  RxUpperLimitStiffness=1e4  RxUpperLimitStiffnessUnits=N*m/deg  RxUpperLimitDamping=10  RxUpperLimitDampingUnits=N*m/(deg/s)  RxUpperLimitTransitionRegionWidth=0.1  RxUpperLimitTransitionRegionWidthUnits=deg  RxTorqueActuationMode=NoTorque  RxMotionActuationMode=ComputedMotion  RxSensePosition=off  RxSenseVelocity=off  RxSenseAcceleration=off  RxSenseTorqueForce=off  RxSenseLowerLimitTorqueForce=off  RxSenseUpperLimitTorqueForce=off  RyPositionTargetSpecify=off  RyPositionTargetPriority=High  RyPositionTargetValue=0  RyPositionTargetValueUnits=deg  RyVelocityTargetSpecify=off  RyVelocityTargetPriority=High  RyVelocityTargetValue=0  RyVelocityTargetValueUnits=deg/s  RyEquilibriumPosition=0  RyEquilibriumPositionUnits=deg  RySpringStiffness=0  RySpringStiffnessUnits=N*m/deg  RyDampingCoefficient=0  RyDampingCoefficientUnits=N*m/(deg/s)  RyLowerLimitSpecify=off  RyLowerLimitBound=-90  RyLowerLimitBoundUnits=deg  RyLowerLimitStiffness=1e4  RyLowerLimitStiffnessUnits=N*m/deg  RyLowerLimitDamping=10  RyLowerLimitDampingUnits=N*m/(deg/s)  RyLowerLimitTransitionRegionWidth=0.1  RyLowerLimitTransitionRegionWidthUnits=deg  RyUpperLimitSpecify=off  RyUpperLimitBound=90  RyUpperLimitBoundUnits=deg  RyUpperLimitStiffness=1e4  RyUpperLimitStiffnessUnits=N*m/deg  RyUpperLimitDamping=10  RyUpperLimitDampingUnits=N*m/(deg/s)  RyUpperLimitTransitionRegionWidth=0.1  RyUpperLimitTransitionRegionWidthUnits=deg  RyTorqueActuationMode=NoTorque  RyMotionActuationMode=ComputedMotion  RySensePosition=off  RySenseVelocity=off  RySenseAcceleration=off  RySenseTorqueForce=off  RySenseLowerLimitTorqueForce=off  RySenseUpperLimitTorqueForce=off  RzPositionTargetSpecify=off  RzPositionTargetPriority=High  RzPositionTargetValue=0  RzPositionTargetValueUnits=deg  RzVelocityTargetSpecify=off  RzVelocityTargetPriority=High  RzVelocityTargetValue=0  RzVelocityTargetValueUnits=deg/s  RzEquilibriumPosition=0  RzEquilibriumPositionUnits=deg  RzSpringStiffness=0  RzSpringStiffnessUnits=N*m/deg  RzDampingCoefficient=0  RzDampingCoefficientUnits=N*m/(deg/s)  RzLowerLimitSpecify=off  RzLowerLimitBound=-90  RzLowerLimitBoundUnits=deg  RzLowerLimitStiffness=1e4  RzLowerLimitStiffnessUnits=N*m/deg  RzLowerLimitDamping=10  RzLowerLimitDampingUnits=N*m/(deg/s)  RzLowerLimitTransitionRegionWidth=0.1  RzLowerLimitTransitionRegionWidthUnits=deg  RzUpperLimitSpecify=off  RzUpperLimitBound=90  RzUpperLimitBoundUnits=deg  RzUpperLimitStiffness=1e4  RzUpperLimitStiffnessUnits=N*m/deg  RzUpperLimitDamping=10  RzUpperLimitDampingUnits=N*m/(deg/s)  RzUpperLimitTransitionRegionWidth=0.1  RzUpperLimitTransitionRegionWidthUnits=deg  RzTorqueActuationMode=NoTorque  RzMotionActuationMode=ComputedMotion  RzSensePosition=off  RzSenseVelocity=off  RzSenseAcceleration=off  RzSenseTorqueForce=off  RzSenseLowerLimitTorqueForce=off  RzSenseUpperLimitTorqueForce=off
  F : PMIOPort  Side=Right
  B : PMIOPort  Port=2  Side=Left
  connections:
  Gimbal HP Spring/LConn1 -- B/RConn1
  Gimbal HP Spring/RConn1 -- F/RConn1

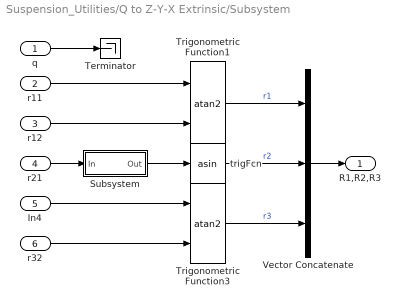
== system Suspension_Utilities/Q to Z-Y-X Extrinsic/Subsystem ==
  q : Inport
  r11 : Inport  Port=2
  r12 : Inport  Port=3
  r21 : Inport  Port=4
  In4 : Inport  Port=5
  r32 : Inport  Port=6
  Subsystem : Subsystem
  Terminator : Terminator
  Trigonometric Function1 : Trigonometry  Operator=atan2
  Trigonometric Function3 : Trigonometry  Operator=atan2
  Vector Concatenate : Concatenate  NumInputs=3
  trigFcn : Trigonometry  Operator=asin
  R1,R2,R3 : Outport  VectorParamsAs1DForOutWhenUnconnected=off
  wires:
  In4/1 -> Trigonometric Function3/1
  Trigonometric Function1/1 -> Vector Concatenate/1  "r1"
  Trigonometric Function3/1 -> Vector Concatenate/3  "r3"
  Subsystem/1(Out) -> trigFcn/1
  q/1 -> Terminator/1
  trigFcn/1 -> Vector Concatenate/2  "r2"
  r32/1 -> Trigonometric Function3/2
  r11/1 -> Trigonometric Function1/1
  r21/1 -> Subsystem/1(In)
  r12/1 -> Trigonometric Function1/2
  Vector Concatenate/1 -> R1,R2,R3/1

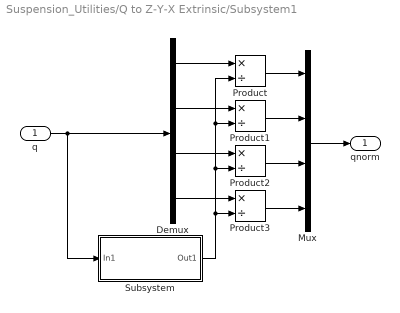
== system Suspension_Utilities/Q to Z-Y-X Extrinsic/Subsystem1 ==
  q : Inport  Unit=1
  Demux : Demux
  Mux : Mux
  Product{,1..3} (4 alike) : Product  Inputs=*/
  Subsystem : Subsystem
  qnorm : Outport  Unit=1  VectorParamsAs1DForOutWhenUnconnected=off
  wires:
  Product1/1 -> Mux/2
  Product3/1 -> Mux/4
  Demux/1 -> Product/1
  Subsystem/1(Out1) -> Product1/2, Product/2, Product2/2, Product3/2
  Mux/1 -> qnorm/1
  Product/1 -> Mux/1
  Demux/3 -> Product2/1
  Demux/4 -> Product3/1
  q/1 -> Demux/1, Subsystem/1(In1)
  Demux/2 -> Product1/1
  Product2/1 -> Mux/3

== system Suspension_Utilities/Shock to Subframe Gimbal/Rigid Gimbal ==
  Gimbal HP Spring : sm_lib/Joints/Gimbal Joint  JointMode=Normal  CompositeWrenchDir=FollowerOnBase  CompositeWrenchFrame=BaseFrame  SenseConstraintForce=off  SenseConstraintTorque=off  SenseTotalForce=off  SenseTotalTorque=off  RxPositionTargetSpecify=on  RxPositionTargetPriority=Low  RxPositionTargetValue=0  RxPositionTargetValueUnits=deg  RxVelocityTargetSpecify=off  RxVelocityTargetPriority=High  RxVelocityTargetValue=0  RxVelocityTargetValueUnits=deg/s  RxEquilibriumPosition=0  RxEquilibriumPositionUnits=deg  RxSpringStiffness=0  RxSpringStiffnessUnits=N*m/deg  RxDampingCoefficient=0  RxDampingCoefficientUnits=N*m/(deg/s)  RxLowerLimitSpecify=off  RxLowerLimitBound=-90  RxLowerLimitBoundUnits=deg  RxLowerLimitStiffness=1e4  RxLowerLimitStiffnessUnits=N*m/deg  RxLowerLimitDamping=10  RxLowerLimitDampingUnits=N*m/(deg/s)  RxLowerLimitTransitionRegionWidth=0.1  RxLowerLimitTransitionRegionWidthUnits=deg  RxUpperLimitSpecify=off  RxUpperLimitBound=90  RxUpperLimitBoundUnits=deg  RxUpperLimitStiffness=1e4  RxUpperLimitStiffnessUnits=N*m/deg  RxUpperLimitDamping=10  RxUpperLimitDampingUnits=N*m/(deg/s)  RxUpperLimitTransitionRegionWidth=0.1  RxUpperLimitTransitionRegionWidthUnits=deg  RxTorqueActuationMode=NoTorque  RxMotionActuationMode=ComputedMotion  RxSensePosition=off  RxSenseVelocity=off  RxSenseAcceleration=off  RxSenseTorqueForce=off  RxSenseLowerLimitTorqueForce=off  RxSenseUpperLimitTorqueForce=off  RyPositionTargetSpecify=off  RyPositionTargetPriority=High  RyPositionTargetValue=0  RyPositionTargetValueUnits=deg  RyVelocityTargetSpecify=off  RyVelocityTargetPriority=High  RyVelocityTargetValue=0  RyVelocityTargetValueUnits=deg/s  RyEquilibriumPosition=0  RyEquilibriumPositionUnits=deg  RySpringStiffness=0  RySpringStiffnessUnits=N*m/deg  RyDampingCoefficient=0  RyDampingCoefficientUnits=N*m/(deg/s)  RyLowerLimitSpecify=off  RyLowerLimitBound=-90  RyLowerLimitBoundUnits=deg  RyLowerLimitStiffness=1e4  RyLowerLimitStiffnessUnits=N*m/deg  RyLowerLimitDamping=10  RyLowerLimitDampingUnits=N*m/(deg/s)  RyLowerLimitTransitionRegionWidth=0.1  RyLowerLimitTransitionRegionWidthUnits=deg  RyUpperLimitSpecify=off  RyUpperLimitBound=90  RyUpperLimitBoundUnits=deg  RyUpperLimitStiffness=1e4  RyUpperLimitStiffnessUnits=N*m/deg  RyUpperLimitDamping=10  RyUpperLimitDampingUnits=N*m/(deg/s)  RyUpperLimitTransitionRegionWidth=0.1  RyUpperLimitTransitionRegionWidthUnits=deg  RyTorqueActuationMode=NoTorque  RyMotionActuationMode=ComputedMotion  RySensePosition=off  RySenseVelocity=off  RySenseAcceleration=off  RySenseTorqueForce=off  RySenseLowerLimitTorqueForce=off  RySenseUpperLimitTorqueForce=off  RzPositionTargetSpecify=off  RzPositionTargetPriority=High  RzPositionTargetValue=0  RzPositionTargetValueUnits=deg  RzVelocityTargetSpecify=off  RzVelocityTargetPriority=High  RzVelocityTargetValue=0  RzVelocityTargetValueUnits=deg/s  RzEquilibriumPosition=0  RzEquilibriumPositionUnits=deg  RzSpringStiffness=0  RzSpringStiffnessUnits=N*m/deg  RzDampingCoefficient=0  RzDampingCoefficientUnits=N*m/(deg/s)  RzLowerLimitSpecify=off  RzLowerLimitBound=-90  RzLowerLimitBoundUnits=deg  RzLowerLimitStiffness=1e4  RzLowerLimitStiffnessUnits=N*m/deg  RzLowerLimitDamping=10  RzLowerLimitDampingUnits=N*m/(deg/s)  RzLowerLimitTransitionRegionWidth=0.1  RzLowerLimitTransitionRegionWidthUnits=deg  RzUpperLimitSpecify=off  RzUpperLimitBound=90  RzUpperLimitBoundUnits=deg  RzUpperLimitStiffness=1e4  RzUpperLimitStiffnessUnits=N*m/deg  RzUpperLimitDamping=10  RzUpperLimitDampingUnits=N*m/(deg/s)  RzUpperLimitTransitionRegionWidth=0.1  RzUpperLimitTransitionRegionWidthUnits=deg  RzTorqueActuationMode=NoTorque  RzMotionActuationMode=ComputedMotion  RzSensePosition=off  RzSenseVelocity=off  RzSenseAcceleration=off  RzSenseTorqueForce=off  RzSenseLowerLimitTorqueForce=off  RzSenseUpperLimitTorqueForce=off
  F : PMIOPort  Side=Right
  B : PMIOPort  Port=2  Side=Left
  connections:
  Gimbal HP Spring/RConn1 -- F/RConn1
  Gimbal HP Spring/LConn1 -- B/RConn1

== system Suspension_Utilities/Wheel Measurements/Calculate Camber ==
  uvec spin axis : Inport
  Demux : Demux  Outputs=3
  Gain : Gain  Gain=-1
  Mux : Mux  Inputs=2
  Trigonometric Function1 : Trigonometry  Operator=atan2
  magnitude : Fcn  Expr=sqrt(u(1)*u(1)+u(2)*u(2))
  Camber : Outport  VectorParamsAs1DForOutWhenUnconnected=off
  wires:
  Demux/1 -> Mux/1
  uvec spin axis/1 -> Demux/1
  Trigonometric Function1/1 -> Camber/1
  Demux/3 -> Gain/1
  Mux/1 -> magnitude/1
  magnitude/1 -> Trigonometric Function1/2
  Demux/2 -> Mux/2
  Gain/1 -> Trigonometric Function1/1

== system Suspension_Utilities/Wheel Measurements/Calculate Camber Z Axis ==
  uvec spin axis : Inport
  Demux : Demux  Outputs=3
  Mux : Mux  Inputs=2
  Trigonometric Function1 : Trigonometry  Operator=atan2
  magnitude : Fcn  Expr=sqrt(u(1)*u(1)+u(2)*u(2))
  Camber : Outport  VectorParamsAs1DForOutWhenUnconnected=off
  wires:
  Demux/2 -> Mux/2
  magnitude/1 -> Trigonometric Function1/2
  Mux/1 -> magnitude/1
  Demux/3 -> Trigonometric Function1/1
  Trigonometric Function1/1 -> Camber/1
  uvec spin axis/1 -> Demux/1
  Demux/1 -> Mux/1

== system Suspension_Utilities/Wheel Measurements/Calculate Toe ==
  uvec spin axis : Inport
  Demux : Demux  Outputs=3
  Gain : Gain
  Gain1 : Gain
  Terminator : Terminator
  Trigonometric Function1 : Trigonometry  Operator=atan2
  Toe : Outport  VectorParamsAs1DForOutWhenUnconnected=off
  wires:
  Demux/2 -> Gain1/1
  uvec spin axis/1 -> Demux/1
  Demux/1 -> Gain/1
  Demux/3 -> Terminator/1
  Gain/1 -> Trigonometric Function1/1
  Gain1/1 -> Trigonometric Function1/2
  Trigonometric Function1/1 -> Toe/1

== system Suspension_Utilities/Wheel Measurements/Calculate Toe X Axis ==
  uvec spin axis : Inport
  Demux : Demux  Outputs=3
  Gain : Gain
  Gain1 : Gain
  Terminator : Terminator
  Trigonometric Function1 : Trigonometry  Operator=atan2
  Toe : Outport  VectorParamsAs1DForOutWhenUnconnected=off
  wires:
  Trigonometric Function1/1 -> Toe/1
  Gain1/1 -> Trigonometric Function1/2
  Gain/1 -> Trigonometric Function1/1
  Demux/3 -> Terminator/1
  Demux/1 -> Gain/1
  uvec spin axis/1 -> Demux/1
  Demux/2 -> Gain1/1

== system Suspension_Utilities/Q to Z-Y-X Extrinsic/Subsystem/Subsystem ==
  In : Inport
  If : If  IfExpression=u1 > 1  ElseIfExpressions=u1 < -1
  If Action Subsystem : sharedtransformsys/Protect asincos input/If Action Subsystem  SystemSampleTime=-1  VariantActivationTime=update diagram  EmptyChoice=off  PassThrough=off  PassThroughVariantControl=(default)  EmptyChoiceVariantControl=(default)  AllowFlexibleInterface=on  Latency=0  AutoFrameSizeCalculation=off
  If Action Subsystem1 : sharedtransformsys/Protect asincos input/If Action Subsystem1  SystemSampleTime=-1  VariantActivationTime=update diagram  EmptyChoice=off  PassThrough=off  PassThroughVariantControl=(default)  EmptyChoiceVariantControl=(default)  AllowFlexibleInterface=on  Latency=0  AutoFrameSizeCalculation=off
  If Action Subsystem2 : sharedtransformsys/Protect asincos input/If Action Subsystem2  SystemSampleTime=-1  VariantActivationTime=update diagram  EmptyChoice=off  PassThrough=off  PassThroughVariantControl=(default)  EmptyChoiceVariantControl=(default)  AllowFlexibleInterface=on  Latency=0  AutoFrameSizeCalculation=off
  Merge : Merge  Inputs=3
  Out : Outport  VectorParamsAs1DForOutWhenUnconnected=off
  wires:
  Merge/1 -> Out/1
  If Action Subsystem/1 -> Merge/1
  If/2 -> If Action Subsystem1/Action
  If Action Subsystem2/1 -> Merge/3
  If/3 -> If Action Subsystem2/Action
  In/1 -> If Action Subsystem2/1, If/1
  If/1 -> If Action Subsystem/Action
  If Action Subsystem1/1 -> Merge/2

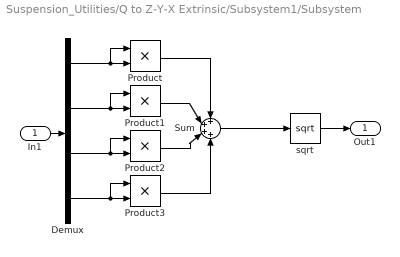
== system Suspension_Utilities/Q to Z-Y-X Extrinsic/Subsystem1/Subsystem ==
  In1 : Inport
  Demux : Demux
  Product{,1..3} (4 alike) : Product
  Sum : Sum  Inputs=4
  sqrt : Sqrt  AlgorithmType=Newton-Raphson
  Out1 : Outport  VectorParamsAs1DForOutWhenUnconnected=off
  wires:
  Demux/4 -> Product3/2, Product3/1
  Product1/1 -> Sum/2
  Demux/3 -> Product2/2, Product2/1
  Product/1 -> Sum/1
  Product2/1 -> Sum/3
  Demux/1 -> Product/2, Product/1
  Demux/2 -> Product1/2, Product1/1
  Product3/1 -> Sum/4
  In1/1 -> Demux/1
  sqrt/1 -> Out1/1
  Sum/1 -> sqrt/1
